simulink model "sistema"  (R2023a)
settings: Solver=ode15s  StartTime=0.0  StopTime=10  MaxStep=1e-2  RelTol=1e-3
libraries: fl_lib x8, nesl_utility x8, ee_lib x6, slpidlib x1
settings Model: Creator=ediel  LastModifiedBy=marti
settings SolverCC: AlgebraicLoopSolver=LineSearch
settings DataIOCC: SaveOutput=off  SignalLogging=off  DSMLogging=off  ReturnWorkspaceOutputs=off  TimeSaveName=t
settings DebuggingCC: AlgebraicLoopMsg=none  ArtificialAlgebraicLoopMsg=none  MaxConsecutiveZCsMsg=none  UnconnectedInputMsg=warning  UnconnectedOutputMsg=warning  UnconnectedLineMsg=warning  ModelReferenceExtraNoncontSigs=none  OperatingPointInterfaceChecksumMismatchMsg=none
settings ModelReferenceCC: EnableRefExpFcnMdlSchedulingChecks=on
settings RTWCC: DLArmComputeVersion=19.05

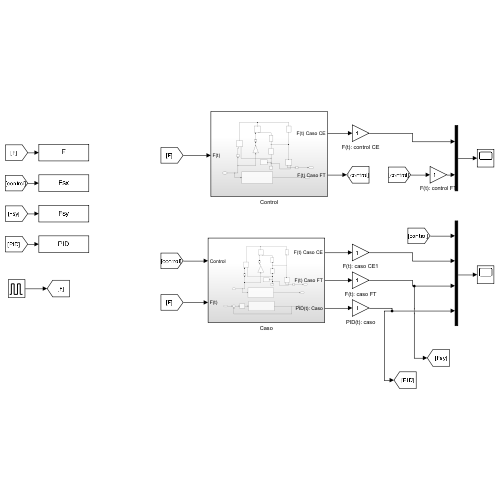
[thumbnail: Simulink's stored preview of the top-level diagram]
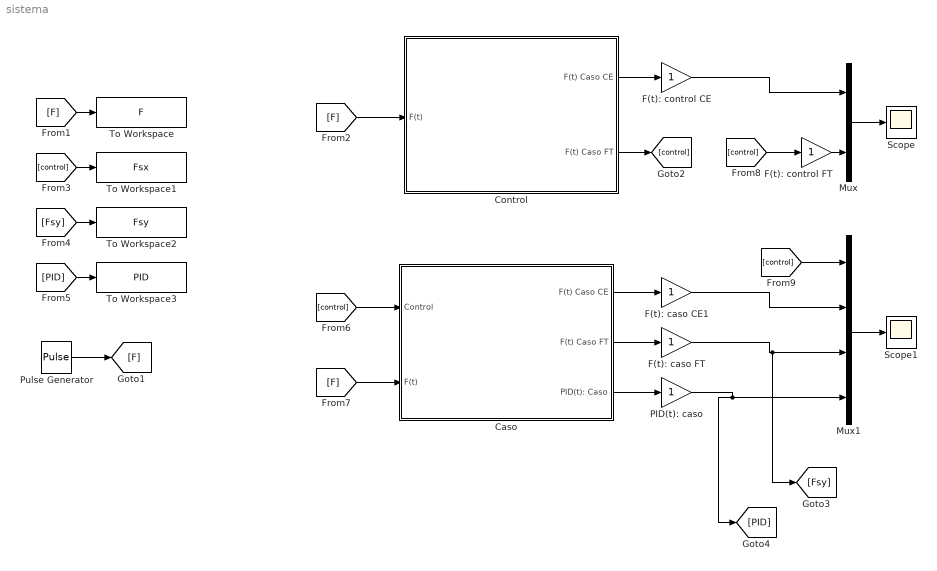
== system sistema ==
  Caso : Subsystem
  Control : Subsystem
  F(t): caso CE1 : Gain
  F(t): caso FT : Gain
  F(t): control CE : Gain
  F(t): control FT : Gain
  Mux : Mux  Inputs=2
  Mux1 : Mux
  PID(t): caso : Gain
  Pulse Generator : DiscretePulseGenerator  PulseType=Time based  Period=10  PulseWidth=10  PhaseDelay=1
  Scope : Scope
  Scope1 : Scope
  To Workspace : ToWorkspace  VariableName=F  SampleTime=-1
  To Workspace1 : ToWorkspace  VariableName=Fsx  SampleTime=-1
  To Workspace2 : ToWorkspace  VariableName=Fsy  SampleTime=-1
  To Workspace3 : ToWorkspace  VariableName=PID  SampleTime=-1
  wires:
  [F] -> To Workspace/1
  [F] -> Control/1(F(t))
  [control] -> To Workspace1/1
  [Fsy] -> To Workspace2/1
  [PID] -> To Workspace3/1
  Pulse Generator/1 -> [F]
  [control] -> Caso/1(Control)
  [F] -> Caso/2(F(t))
  Control/2(F(t) Caso FT) -> [control]
  Control/1(F(t) Caso CE) -> F(t): control CE/1
  Caso/1(F(t) Caso CE) -> F(t): caso CE1/1
  Caso/2(F(t) Caso FT) -> F(t): caso FT/1
  Caso/3(PID(t): Caso) -> PID(t): caso/1
  F(t): control CE/1 -> Mux/1
  [control] -> F(t): control FT/1
  F(t): control FT/1 -> Mux/2
  Mux/1 -> Scope/1
  [control] -> Mux1/1
  F(t): caso CE1/1 -> Mux1/2
  F(t): caso FT/1 -> Mux1/3, [Fsy]
  PID(t): caso/1 -> Mux1/4, [PID]
  Mux1/1 -> Scope1/1

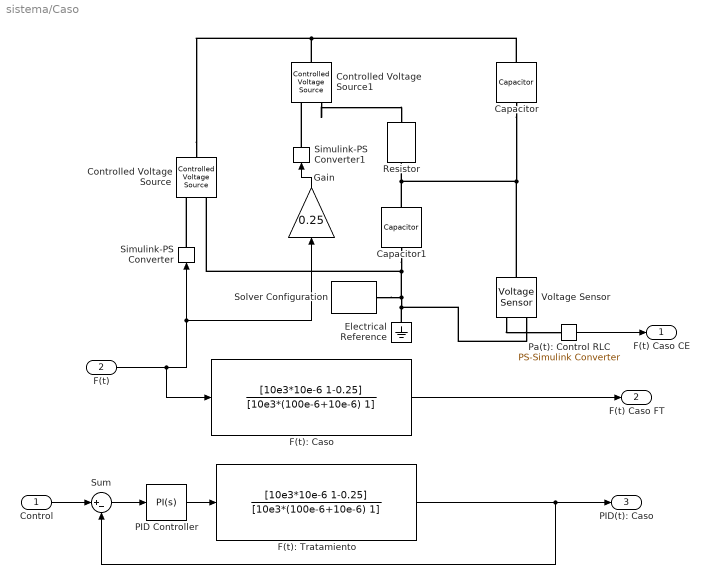
== system sistema/Caso ==
  Control : Inport
  F(t) : Inport  Port=2
  Capacitor : ee_lib/Passive/Capacitor  cap_option=0  c=10 uF  Cvec=[1e-05, 1e-06] F  Vvec=[0, 10] V  CV_table_symmetry=1  f_vec=[1, 10] kHz  DFext_vec=[.8, 1.2]  enable_C_tol=0  averaging_period=0 s  C_tol=5  tol_distribution=1  nSigma=4  r=1e-6 Ohm  g=0 1/Ohm  enable_operating_limits=0  enable_faults=ee.enum.enable.no  fault_action=simscape.enum.assert.action.none  Cscale_faulted=100  R_faulted=1e-3 Ohm  G_faulted=0 1/Ohm  tau_fault=1e-3 s  fault_trigger=ee.enum.faults.faultTrigger.temporal  t_fault=1 s  max_permissible_voltage_range=[-100, 100] V  t_fail_on_voltage=1 s  operating_limit_action=2  max_working_voltage_range=[-25, 25] V  power_rating=1 W  i_specify=off  i_priority=None  i=0 A  i_nominal_specify=off  i_nominal_unit=A  i_nominal_value=1  v_specify=off  v_priority=None  v=0 V  v_nominal_specify=off  v_nominal_unit=V  v_nominal_value=1  vc_specify=off  vc_priority=High  vc=0 V  vc_nominal_specify=off  vc_nominal_unit=V  vc_nominal_value=1
  Capacitor1 : ee_lib/Passive/Capacitor  cap_option=0  c=100 uF  Cvec=[1e-05, 1e-06] F  Vvec=[0, 10] V  CV_table_symmetry=1  f_vec=[1, 10] kHz  DFext_vec=[.8, 1.2]  enable_C_tol=0  averaging_period=0 s  C_tol=5  tol_distribution=1  nSigma=4  r=1e-6 Ohm  g=0 1/Ohm  enable_operating_limits=0  enable_faults=ee.enum.enable.no  fault_action=simscape.enum.assert.action.none  Cscale_faulted=100  R_faulted=1e-3 Ohm  G_faulted=0 1/Ohm  tau_fault=1e-3 s  fault_trigger=ee.enum.faults.faultTrigger.temporal  t_fault=1 s  max_permissible_voltage_range=[-100, 100] V  t_fail_on_voltage=1 s  operating_limit_action=2  max_working_voltage_range=[-25, 25] V  power_rating=1 W  i_specify=off  i_priority=None  i=0 A  i_nominal_specify=off  i_nominal_unit=A  i_nominal_value=1  v_specify=off  v_priority=None  v=0 V  v_nominal_specify=off  v_nominal_unit=V  v_nominal_value=1  vc_specify=off  vc_priority=High  vc=0 V  vc_nominal_specify=off  vc_nominal_unit=V  vc_nominal_value=1
  Controlled Voltage Source : fl_lib/Electrical/Electrical Sources/Controlled Voltage Source
  Controlled Voltage Source1 : fl_lib/Electrical/Electrical Sources/Controlled Voltage Source
  Electrical Reference : fl_lib/Electrical/Electrical Elements/Electrical Reference
  F(t): Caso : TransferFcn  Numerator=[10e3*10e-6 1-0.25]  Denominator=[10e3*(100e-6+10e-6) 1]
  F(t): Tratamiento : TransferFcn  Numerator=[10e3*10e-6 1-0.25]  Denominator=[10e3*(100e-6+10e-6) 1]
  Gain : Gain  Gain=0.25
  PID Controller : slpidlib/PID Controller  Controller=PI  Form=Parallel  TimeDomain=Continuous-time  UseExternalTs=off  SampleTime=-1  IntegratorMethod=Forward Euler  FilterMethod=Forward Euler  ControllerParametersSource=internal  P=0.0214622932954377  I=42283.1371300519  UseKiTs=off  D=0  N=100  UseFilter=on  TunerSelectOption=Transfer Function Based (PID Tuner App)  InitialConditionSource=internal  InitialConditionForIntegrator=0  InitialConditionForFilter=0  DifferentiatorICPrevScaledInput=0  ExternalReset=none  TrackingMode=off  Kt=1  LimitOutput=off  SatLimitsSource=internal  UpperSaturationLimit=inf  LowerSaturationLimit=-inf  LinearizeAsGain=on  AntiWindupMode=none  Kb=1  LimitIntegrator=off  UpperIntegratorSaturationLimit=inf  LowerIntegratorSaturationLimit=-inf  POutMin=[]  POutMax=[]  IOutMin=[]  IOutMax=[]  DOutMin=[]  DOutMax=[]  NOutMin=[]  NOutMax=[]  SumOutMin=[]  SumOutMax=[]  SaturationOutMin=[]  SaturationOutMax=[]  PParamMin=[]  PParamMax=[]  IParamMin=[]  IParamMax=[]  DParamMin=[]  DParamMax=[]  NParamMin=[]  NParamMax=[]  KbParamMin=[]  KbParamMax=[]  KtParamMin=[]  KtParamMax=[]  KbOutMin=[]  KbOutMax=[]  KtOutMin=[]  KtOutMax=[]  IntegratorOutMin=[]  IntegratorOutMax=[]  FilterOutMin=[]  FilterOutMax=[]  SumI1OutMin=[]  SumI1OutMax=[]  SumI2OutMin=[]  SumI2OutMax=[]  SumI3OutMin=[]  SumI3OutMax=[]  SumI4OutMin=[]  SumI4OutMax=[]  SumDOutMin=[]  SumDOutMax=[]  DifferentiatorOutMin=[]  DifferentiatorOutMax=[]  FilterDiffOutCoefMin=[]  FilterDiffOutCoefMax=[]  ReciprocalOutMin=[]  ReciprocalOutMax=[]  SumDenOutMin=[]  SumDenOutMax=[]  SumNumOutMin=[]  SumNumOutMax=[]  DivideOutMin=[]  DivideOutMax=[]  UdiffTsProdOutMin=[]  UdiffTsProdOutMax=[]  NTsProdOutMin=[]  NTsProdOutMax=[]  UintegralTsProdOutMin=[]  UintegralTsProdOutMax=[]  UngainTsProdOutMin=[]  UngainTsProdOutMax=[]  ClampingZeroOutDataTypeStr=Inherit: Inherit via back propagation  ClampingZeroOutMin=[]  ClampingZeroOutMax=[]  FilterDenConstantOutDataTypeStr=Inherit: Inherit via back propagation  FilterDenConstantOutMin=[]  FilterDenConstantOutMax=[]  PCopyOutDataTypeStr=Inherit: Inherit via back propagation  PCopyOutMin=[]  PCopyOutMax=[]  NCopyOutDataTypeStr=Inherit: Inherit via back propagation  NCopyOutMin=[]  NCopyOutMax=[]  IntegratorContinuousStateAttributes=''  IntegratorStateMustResolveToSignalObject=off  IntegratorRTWStateStorageClass=Auto  FilterContinuousStateAttributes=''  FilterStateMustResolveToSignalObject=off  FilterRTWStateStorageClass=Auto  ParallelPVariant=InternalParameters  IdealPVariant=Disabled  IVariant=InternalParameters  DVariant=Disabled  IntegratorVariant=Continuous  SatVariant=Disabled  AWVariant=Passthrough  PCopyVariant=Disabled  TRVariant=Disabled  FdbkBlocksVariant=Forward  IdealPFdbkVariant=Disabled  SatFdbkVariant=Disabled  DerivativeFilterVariant=Disabled  NVariant=Disabled  NCopyVariant=Disabled_SignalSpec  FilterICVariant=Disabled  IntegratorICVariant=InternalICs  ExternalResetVariant=Disabled  TRSumVariant=Passthrough  SumFdbkVariant=Disabled  SumVariant=Sum_PI  TsampFilterVariant=InternalTs  TsampNgainVariant=Passthrough  TsampIntegralVariant=Disabled_SignalSpec  ExternalSaturationOutDataTypeStr=Inherit: Same as second input
  Pa(t): Control RLC : nesl_utility/PS-Simulink Converter  PhysicalDomain=network_engine_domain  SubClassName=ps_output  LeftPortType=input  RightPortType=output  PseudoPeriodic=off  Frequencies=[]  VectorFormat=1-D array  Unit=inherit  AffineConversion=off
  Resistor : ee_lib/Passive/Resistor  R=10 kOhm  enable_R_tol=0  R_tol=5  tol_distribution=1  nSigma=4  enable_operating_limits=0  operating_limit_action=2  power_rating=1 W  max_working_voltage=100 V  enable_faults=ee.enum.enable.no  fault_action=simscape.enum.assert.action.none  R_faulted=inf Ohm  fault_trigger=ee.enum.faults.faultTrigger.temporal  t_fault=1 s  max_permissible_current=1 A  t_fail_on_current=1 s  noise_mode=0  Tdevice=25 degC  sample_time=1e-3 s  repeatability=1  user_seed=0  auto_seed=2619357310  power_derating_T1=70 degC  power_derating_T2=155 degC  operating_temperature_range_vec=[-50, 150] degC  alpha=3.93e-3 1/K  Tmeas=25 degC  thermal_mass=100 J/K  temperature_specify=off  temperature_priority=High  temperature=298.15 K  temperature_nominal_specify=off  temperature_nominal_unit=K  temperature_nominal_value=1
  Simulink-PS Converter : nesl_utility/Simulink-PS Converter  PhysicalDomain=network_engine_domain  SubClassName=ps_input  LeftPortType=input  RightPortType=output  PseudoPeriodic=off  Frequencies=[]  NoiseDistribution=none  NoiseParameters=[]  Unit=1  AffineConversion=off  FilteringAndDerivatives=provide  SimscapeFilterOrder=1  InputFilterTimeConstant=0.001  UdotUserProvided=0
  Simulink-PS Converter1 : nesl_utility/Simulink-PS Converter  PhysicalDomain=network_engine_domain  SubClassName=ps_input  LeftPortType=input  RightPortType=output  PseudoPeriodic=off  Frequencies=[]  NoiseDistribution=none  NoiseParameters=[]  Unit=1  AffineConversion=off  FilteringAndDerivatives=provide  SimscapeFilterOrder=1  InputFilterTimeConstant=0.001  UdotUserProvided=0
  Solver Configuration : nesl_utility/Solver Configuration  PhysicalDomain=network_engine_domain  SubClassName=solver  LeftPortType=input  RightPortType=generic  Tones=[]  Harmonics=[]  SimulateNoise=off  Profile=off  UseLocalSampling=off  EnableSwitchedLinearOptims=on  FrequencyDomain=off  UseCCode=off  RelTol=0.001  AbsTol=1e-06  MinStep=1e-09  ToWorkspace=off  RevertToSquareIcSolve=off  NumHomotopyIterations=100  PhasorMode=off  PhasorModeNumHarmonics=1  ConsistencySolver=NEWTON_FTOL  IndexReductionMethod=DerivativeReplacement  DoDC=off  ResidualTolerance=1e-09  ConsistencyTolSource=GLOBAL  ConsistencyAbsTol=0.001  ConsistencyRelTol=0.001  ConsistencyTolFactor=0.001  UseLocalSolver=off  LocalSolverChoice=NE_BACKWARD_EULER_ADVANCER  ResolveIndetEquations=on  FunctionEvalNumThread=1  LocalSolverSampleTime=0.001  DoFixedCost=off  MaxNonlinIter=3  MaxModeIter=2  ComputeImpulses=off  ImpulseIterations=2  LinearAlgebra=auto  LinearAlgebraNumThread=0  EquationFormulation=NE_TIME_EF  DelaysMemoryBudget=1024  AutomaticFiltering=on  FilteringTimeConstant=0.001  PartitionStorageMethod=AS_NEEDED  PartitionMemoryBudget=1024  PartitionMethod=ROBUST
  Sum : Sum  Inputs=|+-
  Voltage Sensor : fl_lib/Electrical/Electrical Sensors/Voltage Sensor
  F(t) Caso CE : Outport
  F(t) Caso FT : Outport  Port=2
  PID(t): Caso : Outport  Port=3
  wires:
  F(t)/1 -> F(t): Caso/1, Gain/1, Simulink-PS Converter/1
  Gain/1 -> Simulink-PS Converter1/1
  Control/1 -> Sum/1
  PID Controller/1 -> F(t): Tratamiento/1
  Sum/1 -> PID Controller/1
  Pa(t): Control RLC/1 -> F(t) Caso CE/1
  F(t): Caso/1 -> F(t) Caso FT/1
  F(t): Tratamiento/1 -> Sum/2, PID(t): Caso/1
  connections:
  Simulink-PS Converter/RConn1 -- Controlled Voltage Source/RConn1
  Simulink-PS Converter1/RConn1 -- Controlled Voltage Source1/RConn1
  Controlled Voltage Source1/RConn2 -- Resistor/LConn1
  Voltage Sensor/LConn1 -- Resistor/RConn1 -- Capacitor1/LConn1 -- Capacitor/RConn1
  Voltage Sensor/RConn2 -- Electrical Reference/LConn1 -- Solver Configuration/RConn1 -- Capacitor1/RConn1 -- Controlled Voltage Source/RConn2
  Controlled Voltage Source/LConn1 -- Capacitor/LConn1 -- Controlled Voltage Source1/LConn1
  Voltage Sensor/RConn1 -- Pa(t): Control RLC/LConn1

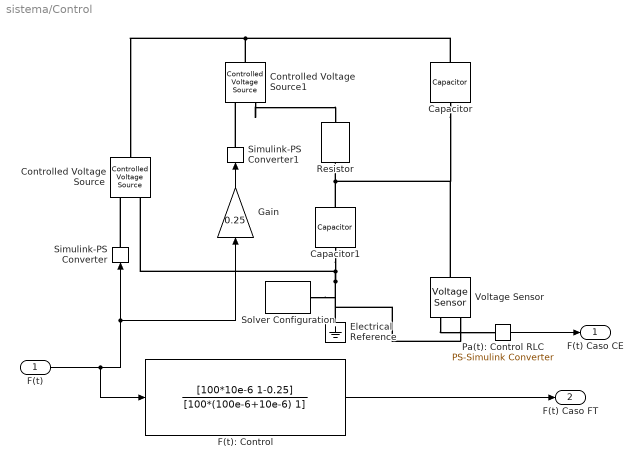
== system sistema/Control ==
  F(t) : Inport
  Capacitor : ee_lib/Passive/Capacitor  cap_option=0  c=10 uF  Cvec=[1e-05, 1e-06] F  Vvec=[0, 10] V  CV_table_symmetry=1  f_vec=[1, 10] kHz  DFext_vec=[.8, 1.2]  enable_C_tol=0  averaging_period=0 s  C_tol=5  tol_distribution=1  nSigma=4  r=1e-6 Ohm  g=0 1/Ohm  enable_operating_limits=0  enable_faults=ee.enum.enable.no  fault_action=simscape.enum.assert.action.none  Cscale_faulted=100  R_faulted=1e-3 Ohm  G_faulted=0 1/Ohm  tau_fault=1e-3 s  fault_trigger=ee.enum.faults.faultTrigger.temporal  t_fault=1 s  max_permissible_voltage_range=[-100, 100] V  t_fail_on_voltage=1 s  operating_limit_action=2  max_working_voltage_range=[-25, 25] V  power_rating=1 W  i_specify=off  i_priority=None  i=0 A  i_nominal_specify=off  i_nominal_unit=A  i_nominal_value=1  v_specify=off  v_priority=None  v=0 V  v_nominal_specify=off  v_nominal_unit=V  v_nominal_value=1  vc_specify=off  vc_priority=High  vc=0 V  vc_nominal_specify=off  vc_nominal_unit=V  vc_nominal_value=1
  Capacitor1 : ee_lib/Passive/Capacitor  cap_option=0  c=100 uF  Cvec=[1e-05, 1e-06] F  Vvec=[0, 10] V  CV_table_symmetry=1  f_vec=[1, 10] kHz  DFext_vec=[.8, 1.2]  enable_C_tol=0  averaging_period=0 s  C_tol=5  tol_distribution=1  nSigma=4  r=1e-6 Ohm  g=0 1/Ohm  enable_operating_limits=0  enable_faults=ee.enum.enable.no  fault_action=simscape.enum.assert.action.none  Cscale_faulted=100  R_faulted=1e-3 Ohm  G_faulted=0 1/Ohm  tau_fault=1e-3 s  fault_trigger=ee.enum.faults.faultTrigger.temporal  t_fault=1 s  max_permissible_voltage_range=[-100, 100] V  t_fail_on_voltage=1 s  operating_limit_action=2  max_working_voltage_range=[-25, 25] V  power_rating=1 W  i_specify=off  i_priority=None  i=0 A  i_nominal_specify=off  i_nominal_unit=A  i_nominal_value=1  v_specify=off  v_priority=None  v=0 V  v_nominal_specify=off  v_nominal_unit=V  v_nominal_value=1  vc_specify=off  vc_priority=High  vc=0 V  vc_nominal_specify=off  vc_nominal_unit=V  vc_nominal_value=1
  Controlled Voltage Source : fl_lib/Electrical/Electrical Sources/Controlled Voltage Source
  Controlled Voltage Source1 : fl_lib/Electrical/Electrical Sources/Controlled Voltage Source
  Electrical Reference : fl_lib/Electrical/Electrical Elements/Electrical Reference
  F(t): Control : TransferFcn  Numerator=[100*10e-6 1-0.25]  Denominator=[100*(100e-6+10e-6) 1]
  Gain : Gain  Gain=0.25
  Pa(t): Control RLC : nesl_utility/PS-Simulink Converter  PhysicalDomain=network_engine_domain  SubClassName=ps_output  LeftPortType=input  RightPortType=output  PseudoPeriodic=off  Frequencies=[]  VectorFormat=1-D array  Unit=inherit  AffineConversion=off
  Resistor : ee_lib/Passive/Resistor  R=100 Ohm  enable_R_tol=0  R_tol=5  tol_distribution=1  nSigma=4  enable_operating_limits=0  operating_limit_action=2  power_rating=1 W  max_working_voltage=100 V  enable_faults=ee.enum.enable.no  fault_action=simscape.enum.assert.action.none  R_faulted=inf Ohm  fault_trigger=ee.enum.faults.faultTrigger.temporal  t_fault=1 s  max_permissible_current=1 A  t_fail_on_current=1 s  noise_mode=0  Tdevice=25 degC  sample_time=1e-3 s  repeatability=1  user_seed=0  auto_seed=3499211588  power_derating_T1=70 degC  power_derating_T2=155 degC  operating_temperature_range_vec=[-50, 150] degC  alpha=3.93e-3 1/K  Tmeas=25 degC  thermal_mass=100 J/K  temperature_specify=off  temperature_priority=High  temperature=298.15 K  temperature_nominal_specify=off  temperature_nominal_unit=K  temperature_nominal_value=1
  Simulink-PS Converter : nesl_utility/Simulink-PS Converter  PhysicalDomain=network_engine_domain  SubClassName=ps_input  LeftPortType=input  RightPortType=output  PseudoPeriodic=off  Frequencies=[]  NoiseDistribution=none  NoiseParameters=[]  Unit=1  AffineConversion=off  FilteringAndDerivatives=provide  SimscapeFilterOrder=1  InputFilterTimeConstant=0.001  UdotUserProvided=0
  Simulink-PS Converter1 : nesl_utility/Simulink-PS Converter  PhysicalDomain=network_engine_domain  SubClassName=ps_input  LeftPortType=input  RightPortType=output  PseudoPeriodic=off  Frequencies=[]  NoiseDistribution=none  NoiseParameters=[]  Unit=1  AffineConversion=off  FilteringAndDerivatives=provide  SimscapeFilterOrder=1  InputFilterTimeConstant=0.001  UdotUserProvided=0
  Solver Configuration : nesl_utility/Solver Configuration  PhysicalDomain=network_engine_domain  SubClassName=solver  LeftPortType=input  RightPortType=generic  Tones=[]  Harmonics=[]  SimulateNoise=off  Profile=off  UseLocalSampling=off  EnableSwitchedLinearOptims=on  FrequencyDomain=off  UseCCode=off  RelTol=0.001  AbsTol=1e-06  MinStep=1e-09  ToWorkspace=off  RevertToSquareIcSolve=off  NumHomotopyIterations=100  PhasorMode=off  PhasorModeNumHarmonics=1  ConsistencySolver=NEWTON_FTOL  IndexReductionMethod=DerivativeReplacement  DoDC=off  ResidualTolerance=1e-09  ConsistencyTolSource=GLOBAL  ConsistencyAbsTol=0.001  ConsistencyRelTol=0.001  ConsistencyTolFactor=0.001  UseLocalSolver=off  LocalSolverChoice=NE_BACKWARD_EULER_ADVANCER  ResolveIndetEquations=on  FunctionEvalNumThread=1  LocalSolverSampleTime=0.001  DoFixedCost=off  MaxNonlinIter=3  MaxModeIter=2  ComputeImpulses=off  ImpulseIterations=2  LinearAlgebra=auto  LinearAlgebraNumThread=0  EquationFormulation=NE_TIME_EF  DelaysMemoryBudget=1024  AutomaticFiltering=on  FilteringTimeConstant=0.001  PartitionStorageMethod=AS_NEEDED  PartitionMemoryBudget=1024  PartitionMethod=ROBUST
  Voltage Sensor : fl_lib/Electrical/Electrical Sensors/Voltage Sensor
  F(t) Caso CE : Outport
  F(t) Caso FT : Outport  Port=2
  wires:
  F(t)/1 -> F(t): Control/1, Gain/1, Simulink-PS Converter/1
  Gain/1 -> Simulink-PS Converter1/1
  Pa(t): Control RLC/1 -> F(t) Caso CE/1
  F(t): Control/1 -> F(t) Caso FT/1
  connections:
  Simulink-PS Converter/RConn1 -- Controlled Voltage Source/RConn1
  Simulink-PS Converter1/RConn1 -- Controlled Voltage Source1/RConn1
  Controlled Voltage Source1/RConn2 -- Resistor/LConn1
  Capacitor1/LConn1 -- Voltage Sensor/LConn1 -- Capacitor/RConn1 -- Resistor/RConn1
  Capacitor1/RConn1 -- Voltage Sensor/RConn2 -- Electrical Reference/LConn1 -- Solver Configuration/RConn1 -- Controlled Voltage Source/RConn2
  Capacitor/LConn1 -- Controlled Voltage Source1/LConn1 -- Controlled Voltage Source/LConn1
  Voltage Sensor/RConn1 -- Pa(t): Control RLC/LConn1
